simulink model "FOCwithLOAD"  (R2024b)
settings: Solver=FixedStepDiscrete  StartTime=0.0  StopTime=inf  RelTol=1e-3
PreLoadFcn:
  | % 自动加载同目录下的 linear_data.m，确保换机/首次打开可直接更新与编译
  | if ~evalin('base', 'exist(''Ts'',''var'') && exist(''pmsm'',''var'') && exist(''SMRC_I_Vsat_thresh'',''var'')')
  |     mdlDir_ = '';
  |     if bdIsLoaded('FOCwithLOAD'), mdlDir_ = fileparts(get_param('FOCwithLOAD', 'FileName')); end
  |     if isempty(mdlDir_), mdlDir_ = fileparts(which('FOCwithLOAD')); end
  |     if isempty(mdlDir_), mdlDir_ = pwd; end
  |     dataFile_ = fullfile(mdlDir_, 'linear_data.m');
  |     if isfile(dataFile_)
  |         assignin('base', 'linearDataFileTmp_', dataFile_);
  |         evalin('base', 'run(linearDataFileTmp_); clear linearDataFileTmp_');
  |     end
  |     clear mdlDir_ dataFile_
  | end
InitFcn:
  | % 自动加载同目录下的 linear_data.m，确保换机/首次打开可直接更新与编译
  | if ~evalin('base', 'exist(''Ts'',''var'') && exist(''pmsm'',''var'') && exist(''SMRC_I_Vsat_thresh'',''var'')')
  |     mdlDir_ = '';
  |     if bdIsLoaded('FOCwithLOAD'), mdlDir_ = fileparts(get_param('FOCwithLOAD', 'FileName')); end
  |     if isempty(mdlDir_), mdlDir_ = fileparts(which('FOCwithLOAD')); end
  |     if isempty(mdlDir_), mdlDir_ = pwd; end
  |     dataFile_ = fullfile(mdlDir_, 'linear_data.m');
  |     if isfile(dataFile_)
  |         assignin('base', 'linearDataFileTmp_', dataFile_);
  |         evalin('base', 'run(linearDataFileTmp_); clear linearDataFileTmp_');
  |     end
  |     clear mdlDir_ dataFile_
  | end
values from neighbouring files (symbols this model uses):
  a_hat = Kt_eff / (pmsm.J * omega_pu_base)    [linear_data.m]
  ADRC_B0 = 6055    [linear_data.m]
  ADRC_Wc = 3.2e-3    (= 0.0032)    [linear_data.m]
  ADRC_Wo = 30    [linear_data.m]
  alpha_ppc = exp(-lambda_ppc*Ts_speed)    [linear_data.m]
  b_hat = pmsm.B/pmsm.J    [linear_data.m]
  beta1 = single(2.0 * w_o)    [linear_data.m]
  beta2_sat_scale = 0.2    [linear_data.m]
  dataType = 'single'    [linear_data.m]
  gamma_reset = 0.9    [linear_data.m]
  inv_a_hat = 1/double(a_hat)    [linear_data.m]
  k_xi = 55    [linear_data.m]
  Kff = 0.98931745    [linear_data.m]
  lambda_ppc = 45    [linear_data.m]
  P_inf_const = 0.004    [linear_data.m]
  PI_params = mcb_SetControllerParameters(pmsm,inverter,PU_System,T_pwm,Ts,Ts_speed)    [linear_data.m]
  pmsm2 = pmsm    [linear_data.m]
  s_limit_sat = 0.9    [linear_data.m]
  speedRPM2mmps = pmlsm.mmps_per_rpm    [linear_data.m]
  target = mcb_SetProcessorDetails('F28379D',PWM_frequency)    [linear_data.m]
  Ts = T_pwm    (= 5e-05)    [linear_data.m]
  Ts_motor = T_pwm/2    (= 2.5e-05)    [linear_data.m]
  Ts_speed = 1*Ts    (= 5e-05)    [linear_data.m]
  w_o = single(200.0)    [linear_data.m]
  z2_limit = single(100.0)    [linear_data.m]
undefined symbols (not defined in the file or in its folder): DiscIntNeverNeededParam, Down, GPTRIP1SEL, GPTRIP2SEL, innerPI, inverter, inverter2, outerPI, pmlsm, pmsm, Tctr, TZ1, TZ2, Up
libraries: c2802xlib x13, simulink x10, c2837xDlib x6, c280xlib x6, slpidlib x5, svdschedulerlib x4, mcbcontrolslib x4, mcbpositiondecoderlib x2, mcbpmsmnonlinearlib x2, autolibpmsmexterior x2, mcbplantlib x2, svdutilitieslib x1
(part 4 of 5)

== system FOCwithLOAD/Motor1 Speed control/Control_System/Closed Loop Control1/Controller ==
  iD_fdbk : Inport
  iQ_fdbk : Inport  Port=2
  IdqRef : Inport  Port=3
  dx_mm : Inport  Port=4
  EnSMRC_I : Inport  Port=5
  AlignModeReadQ : DataStoreRead  DataStoreName=AlignMode  IndexOptions=Index vector (dialog)  Indices=1  OutputSizes=1
  Demux : Demux  Outputs=2
  Inner D axis Controller : Subsystem
  Inner Q axis Controller : Subsystem
  IqFdbkAlignSw : Switch  Criteria=u2 > Threshold  Threshold=0.5  SaturateOnIntegerOverflow=off  InputSameDT=off
  VqAlignSw : Switch  Criteria=u2 > Threshold  Threshold=0.5  SaturateOnIntegerOverflow=off  InputSameDT=off
  ZeroSingleQ : Constant  Value=0  OutDataTypeStr=single
  uD_req : Outport
  uQ_req : Outport  Port=2
  wires:
  iD_fdbk/1 -> Inner D axis Controller/2(iD_fdbk)
  IdqRef/1 -> Demux/1
  Demux/1 -> Inner D axis Controller/1(iD_req)
  Demux/2 -> Inner Q axis Controller/1(iQ_req)
  Inner D axis Controller/1(uD_req) -> uD_req/1  "uD_req"
  VqAlignSw/1 -> uQ_req/1
  Inner Q axis Controller/1(uQ_req) -> VqAlignSw/3  "uQ_req"
  IqFdbkAlignSw/1 -> Inner Q axis Controller/2(iQ_fdbk)
  iQ_fdbk/1 -> IqFdbkAlignSw/3
  AlignModeReadQ/1 -> IqFdbkAlignSw/2, VqAlignSw/2
  ZeroSingleQ/1 -> IqFdbkAlignSw/1, VqAlignSw/1

== system FOCwithLOAD/Motor1 Speed control/Control_System/Closed Loop Control1/SVPWM ==
  note: 零序分量注入
  u_alpha : Inport
  u_beta : Inport  Port=2
  VBus : Inport  Port=3
  Constant : Constant
  Constant3 : Constant  Commented=on  Value=0.5  OutDataTypeStr=single
  Divide1 : Product  Commented=on  Inputs=*/
  Gain : Gain  Gain=2/Ts
  InvClark : Subsystem  Commented=on
  Scope : Scope
  Scope1 : Scope
  Sector Caculate : Subsystem
  Subtract : Sum  Inputs=+-  OutDataTypeStr=single
  Sum : Sum  Commented=on  Inputs=++|
  Sum2 : Sum  Commented=on  Inputs=|++
  T1T1 Caculate : Subsystem
  Tcm Caculate : Subsystem
  Tpwm : Constant  Value=Ts  OutDataTypeStr=double
  XYZ Caculate : Subsystem
  ei_t : Subsystem  Commented=on
  DutyABC : Outport
  wires:
  Constant3/1 -> Sum2/2
  Divide1/1 -> Sum2/1
  InvClark/1(u_abc_spwm) -> ei_t/1(u_abc_spwm), Sum/2  "spwm"
  ei_t/1(sit) -> Sum/1  "eit"
  Sum/1 -> Divide1/1
  u_beta/1 -> InvClark/2(u_beta), XYZ Caculate/2(Ubeta), Sector Caculate/2(Ubeta)
  u_alpha/1 -> InvClark/1(u_alpha), Sector Caculate/1(Ualpha), XYZ Caculate/1(Ualpha)
  VBus/1 -> XYZ Caculate/4(Udc), Divide1/2
  Constant/1 -> Subtract/1
  Tcm Caculate/1(Tcm1 Tcm2 Tcm3) -> Scope1/1, Gain/1
  T1T1 Caculate/2(T2) -> Tcm Caculate/3(T2)
  XYZ Caculate/1(XYZ) -> T1T1 Caculate/2(XYZ)
  Gain/1 -> Subtract/2
  Sector Caculate/1("N ") -> Tcm Caculate/1(N), T1T1 Caculate/1(N)
  Tpwm/1 -> XYZ Caculate/3(Ts), Tcm Caculate/4(Tpwm), T1T1 Caculate/3(Tpwm)
  T1T1 Caculate/1(T1) -> Tcm Caculate/2(T1)
  Subtract/1 -> DutyABC/1, Scope/1

== system FOCwithLOAD/Motor1 Speed control/Control_System/Closed Loop Control1/Sample Choice ==
  note: 在电流采样中，ADC在mosfet导通时，进行电压测算，反推出电流，
      | 当上桥臂极高占空比时，导致下桥臂占空比极低，测量时间极短。
      | 开关噪声等会影响测量。
      |
      | 判断占空比大小，选用合适的下桥臂电流进行计算。Ia+Ib+Ic=0
  Duty : Inport
  Iabc : Inport  Port=2
  AB 采样计算2 : Subsystem  TreatAsAtomicUnit=on
  AC 采样计算1 : Subsystem  TreatAsAtomicUnit=on
  BC 采样计算 : Subsystem  TreatAsAtomicUnit=on
  Demux1 : Demux  Outputs=3
  If : If  NumInputs=3  IfExpression=u1 >= u2 & u1 >= u3  ElseIfExpressions=u2 >= u1 & u2 >= u3
  Merge : Merge  Inputs=3
  IABC : Outport
  wires:
  If/1 -> BC 采样计算/Action  "BC采样"
  Iabc/1 -> BC 采样计算/1(Iabc), AB 采样计算2/1(Iabc), AC 采样计算1/1(Iabc)
  If/2 -> AC 采样计算1/Action  "AC采样"
  Duty/1 -> Demux1/1
  Demux1/1 -> If/1
  If/3 -> AB 采样计算2/Action  "AB采样"
  Merge/1 -> IABC/1
  BC 采样计算/1(IABC) -> Merge/1
  Demux1/3 -> If/3
  Demux1/2 -> If/2
  AC 采样计算1/1(IABC) -> Merge/2
  AB 采样计算2/1(IABC) -> Merge/3

== system FOCwithLOAD/Motor1 Speed control/Control_System/Closed Loop Control1/clark ==
  note: $i_\alpha=\frac{2}{3}i_a-\frac{1}{3}(i_b+i_c) \\ i_\beta=\frac{\sqrt{3}}{3}(i_b-i_c)$
  i_a : Inport
  i_b : Inport  Port=2
  i_c : Inport  Port=3
  Gain : Gain  Gain=2/3
  Gain1 : Gain  Gain=1/3
  Gain2 : Gain  Gain=sqrt(3)/3
  Sum : Sum  Inputs=|++
  Sum1 : Sum  Inputs=|+-
  Sum2 : Sum  Inputs=+-|
  i_alpha : Outport
  i_beta : Outport  Port=2
  wires:
  Gain2/1 -> i_beta/1
  Sum2/1 -> Gain2/1
  Sum1/1 -> i_alpha/1
  Gain1/1 -> Sum1/2
  Gain/1 -> Sum1/1
  i_a/1 -> Gain/1
  i_c/1 -> Sum/2, Sum2/2
  Sum/1 -> Gain1/1
  i_b/1 -> Sum/1, Sum2/1

== system FOCwithLOAD/Motor1 Speed control/Control_System/Closed Loop Control1/inv_park ==
  note: $i_{\alpha} = i_d cos(\theta_e )- i_q sin(\theta_e )\\ i_{\beta} = i_d sin(\theta_e )+ i_q cos(\theta_e )$
  u_d : Inport
  u_q : Inport  Port=2
  sincos : Inport  Port=3
  Add : Sum  Inputs=+-
  Add1 : Sum
  Demux : Demux  Outputs=2
  Product{,1..3} (4 alike) : Product
  u_alpha : Outport
  u_beta : Outport  Port=2
  wires:
  sincos/1 -> Demux/1
  Demux/2 -> Product3/2, Product/2
  Demux/1 -> Product2/2, Product1/2
  Add1/1 -> u_beta/1
  Product3/1 -> Add1/2
  Product2/1 -> Add1/1
  Add/1 -> u_alpha/1
  Product1/1 -> Add/2
  u_q/1 -> Product1/1, Product3/1
  Product/1 -> Add/1
  u_d/1 -> Product/1, Product2/1  "i_d"

== system FOCwithLOAD/Motor1 Speed control/Control_System/Closed Loop Control1/park ==
  note: $i_{d} = i_{\alpha} cos(\theta_e )+ i_{\beta} sin(\theta_e ) \\ i_{q} = -i_{\alpha} sin(\theta_e )+ i_{\beta} cos(\theta_e )$
  i_alpha : Inport
  i_beta : Inport  Port=2
  sincos : Inport  Port=3
  Demux : Demux  Outputs=2
  Product{,1..3} (4 alike) : Product
  Sum : Sum  Inputs=|++
  Sum1 : Sum  Inputs=|-+
  i_d : Outport
  i_q : Outport  Port=2
  wires:
  sincos/1 -> Demux/1
  Sum1/1 -> i_q/1
  Product3/1 -> Sum1/2
  Product2/1 -> Sum1/1
  i_beta/1 -> Product1/1, Product3/1
  Sum/1 -> i_d/1
  Product1/1 -> Sum/2
  Product/1 -> Sum/1
  Demux/1 -> Product2/2, Product1/2  "sin"
  Demux/2 -> Product/2, Product3/2  "cos"
  i_alpha/1 -> Product/1, Product2/1

== system FOCwithLOAD/Motor1 Speed control/Input Scaling/ Calculate Position and Speed/PosDelta ==
  theta_pu : Inport
  C_Half : Constant  Value=single(0.5)
  C_InitOne : Constant  Value=single(1.0)
  C_One : Constant  Value=single(1.0)
  C_Zero : Constant  Value=single(0.0)
  Gain_mm : Gain  Gain=single(20.0)
  Mod_Wrap : Math  Operator=mod
  Sum_AddHalf : Sum
  Sum_Diff : Sum  Inputs=+-
  Sum_SubHalf : Sum  Inputs=+-
  Sw_Init : Switch  Criteria=u2 > Threshold  Threshold=0.5  SaturateOnIntegerOverflow=off  InputSameDT=off
  ToSingle : DataTypeConversion  OutDataTypeStr=single  SaturateOnIntegerOverflow=off  RndMeth=Floor
  UD_Init : UnitDelay  InitialCondition=single(0.0)  SampleTime=-1  HasFrameUpgradeWarning=on
  UD_Theta : UnitDelay  InitialCondition=single(0)  SampleTime=-1  HasFrameUpgradeWarning=on
  dx_mm : Outport
  wires:
  Sw_Init/1 -> dx_mm/1
  C_Zero/1 -> Sw_Init/3
  UD_Init/1 -> Sw_Init/2
  Gain_mm/1 -> Sw_Init/1
  C_InitOne/1 -> UD_Init/1
  Sum_SubHalf/1 -> Gain_mm/1
  Mod_Wrap/1 -> Sum_SubHalf/1
  C_One/1 -> Mod_Wrap/2
  Sum_AddHalf/1 -> Mod_Wrap/1
  C_Half/1 -> Sum_AddHalf/2, Sum_SubHalf/2
  Sum_Diff/1 -> Sum_AddHalf/1
  UD_Theta/1 -> Sum_Diff/2
  ToSingle/1 -> UD_Theta/1, Sum_Diff/1
  theta_pu/1 -> ToSingle/1

== system FOCwithLOAD/Motor1 Speed control/Input Scaling/Calculate Phase Currents/Data_Type ==
  In1 : Inport
  Data_Type_Fixed_Point : Subsystem  VariantControl=~isequal(dataType,'single')
  Data_Type_Float : Subsystem  VariantControl=isequal(dataType,'single')
  Iabc_meas_Real : Outport

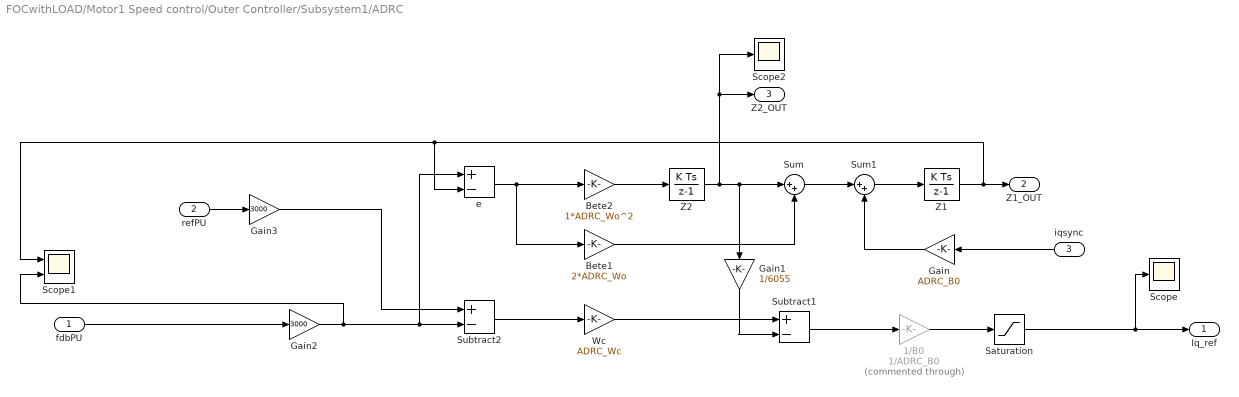
== system FOCwithLOAD/Motor1 Speed control/Outer Controller/Subsystem1/ADRC ==
  fdbPU : Inport
  refPU : Inport  Port=2
  iqsync : Inport  Port=3
  1/B0 : Gain  Commented=through  Gain=1/ADRC_B0
  Bete1 : Gain  Gain=2*ADRC_Wo
  Bete2 : Gain  Gain=1*ADRC_Wo^2
  Gain : Gain  Gain=ADRC_B0
  Gain1 : Gain  Gain=1/6055
  Gain2 : Gain  Gain=3000
  Gain3 : Gain  Gain=3000
  Saturation : Saturate  UpperLimit=8  LowerLimit=-8
  Scope : Scope
  Scope1 : Scope  NumInputPorts=2
  Scope2 : Scope
  Subtract1 : Sum  Inputs=+-
  Subtract2 : Sum  Inputs=+-
  Sum : Sum  Inputs=|++
  Sum1 : Sum  Inputs=|++
  Wc : Gain  Gain=ADRC_Wc
  Z1 : DiscreteIntegrator  SampleTime=-1  ICPrevOutput=DiscIntNeverNeededParam  ICPrevScaledInput=DiscIntNeverNeededParam
  Z2 : DiscreteIntegrator  SampleTime=-1  ICPrevOutput=DiscIntNeverNeededParam  ICPrevScaledInput=DiscIntNeverNeededParam
  e : Sum  Inputs=+-
  Iq_ref : Outport
  Z1_OUT : Outport  Port=2
  Z2_OUT : Outport  Port=3
  wires:
  e/1 -> Bete1/1, Bete2/1
  Bete2/1 -> Z2/1
  Bete1/1 -> Sum/2
  Sum/1 -> Sum1/1
  Wc/1 -> Subtract1/1
  Subtract2/1 -> Wc/1
  Subtract1/1 -> 1/B0/1
  1/B0/1 -> Saturation/1
  Z2/1 -> Scope2/1, Z2_OUT/1, Sum/1, Gain1/1
  Sum1/1 -> Z1/1
  Z1/1 -> Z1_OUT/1, e/2, Scope1/1
  Saturation/1 -> Scope/1, Iq_ref/1
  iqsync/1 -> Gain/1
  refPU/1 -> Gain3/1
  Gain/1 -> Sum1/2
  Gain1/1 -> Subtract1/2
  Gain2/1 -> Scope1/2, e/1, Subtract2/2
  Gain3/1 -> Subtract2/1
  fdbPU/1 -> Gain2/1

== system FOCwithLOAD/Motor1 Speed control/Outer Controller/ppc/P_decay ==
  P_inf_const : Inport
  P_select : Inport  Port=2
  1 : Sum  Inputs=|++
  P_z1 : UnitDelay  SampleTime=-1  HasFrameUpgradeWarning=on
  PminusPinf : Sum  Inputs=|+-
  alpha_gain : Gain  Gain=alpha_ppc
  P_decay_sum : Outport
  wires:
  P_inf_const/1 -> PminusPinf/2, 1/2
  P_select/1 -> P_z1/1
  alpha_gain/1 -> 1/1
  1/1 -> P_decay_sum/1
  P_z1/1 -> PminusPinf/1
  PminusPinf/1 -> alpha_gain/1

== system FOCwithLOAD/Motor1 Speed control/Outer Controller/ppc/P_reset ==
  e_calc : Inport
  P_inf_const : Inport  Port=2
  Gain : Gain  Gain=1.25
  P_floor_sum : Sum  Inputs=|++
  P_reset_max : MinMax  Function=max  Inputs=2
  abs_e : Abs  SaturateOnIntegerOverflow=off
  eps_p_const : Constant  Value=0.001
  P_reset : Outport
  wires:
  P_floor_sum/1 -> P_reset_max/2
  abs_e/1 -> Gain/1
  eps_p_const/1 -> P_floor_sum/2
  Gain/1 -> P_reset_max/1
  P_reset_max/1 -> P_reset/1
  e_calc/1 -> abs_e/1
  P_inf_const/1 -> P_floor_sum/1

== system FOCwithLOAD/Motor1 Speed control/Outer Controller/ppc/eso ==
  Iq_ref_prev : Inport
  speed_fdbk : Inport  Port=2
  Abs : Abs  SaturateOnIntegerOverflow=off
  Compare To Constant : simulink/Logic and Bit Operations/Compare To Constant  relop=>  const=7.95  OutDataTypeStr=boolean
  Constant : Constant  Value=w_o * w_o
  Constant1 : Constant  Value=beta2_sat_scale * w_o * w_o
  Discrete-Time Integrator1 : DiscreteIntegrator  SampleTime=-1  ICPrevOutput=DiscIntNeverNeededParam  ICPrevScaledInput=DiscIntNeverNeededParam
  Gain1 : Gain  Gain=a_hat
  Gain2 : Gain  Gain=-beta1
  Gain3 : Gain  Gain=-b_hat
  Gain4 : Gain  Gain=-1
  Gain5 : Gain  Gain=Ts_speed
  Product : Product
  Saturation : Saturate  UpperLimit=z2_limit  LowerLimit=-z2_limit
  Sum : Sum  Inputs=++++
  Switch : Switch  Criteria=u2 ~= 0  SaturateOnIntegerOverflow=off  InputSameDT=off
  Unit Delay : UnitDelay  SampleTime=-1  HasFrameUpgradeWarning=on
  e : Sum  Inputs=|++
  e_obs : Sum  Inputs=|+-
  Z1 : Outport
  Z2 : Outport  Port=2
  wires:
  speed_fdbk/1 -> e_obs/2
  e_obs/1 -> Product/2, Gain2/1  "e_obs"
  Saturation/1 -> Sum/1, Z2/1, Unit Delay/1  "z2_next"
  Iq_ref_prev/1 -> Abs/1, Gain1/1
  Gain1/1 -> Sum/2
  Gain2/1 -> Sum/3
  Sum/1 -> Discrete-Time Integrator1/1
  Discrete-Time Integrator1/1 -> Gain3/1, Z1/1, e_obs/1
  Gain3/1 -> Sum/4
  Abs/1 -> Compare To Constant/1
  Compare To Constant/1 -> Switch/2
  Constant1/1 -> Switch/1
  Constant/1 -> Switch/3
  Product/1 -> Gain4/1
  Switch/1 -> Product/1
  Gain4/1 -> Gain5/1
  Gain5/1 -> e/1
  e/1 -> Saturation/1
  Unit Delay/1 -> e/2

== system FOCwithLOAD/Motor1 Speed control/Outer Controller/ppc/ref_jump_detect ==
  SpeedPU_req : Inport
  e__calc : Inport  Port=2
  p_select : Inport  Port=3
  Abs : Abs  SaturateOnIntegerOverflow=off
  Delay : Delay  DelayLength=1  InitialCondition=0
  Gain1 : Gain  Gain=gamma_reset
  GreaterThan : RelationalOperator  Operator=>  OutDataTypeStr=boolean  RndMeth=Simplest  InputSameDT=off
  Logical Operator : Logic  Operator=OR  AllPortsSameDT=off  OutDataTypeStr=boolean
  abs_dwref : Abs  SaturateOnIntegerOverflow=off
  delta_ref_const : Constant  Value=P_inf_const
  dwref_calc : Sum  Inputs=|+-
  ref_jump_detect : RelationalOperator  Operator=>  OutDataTypeStr=boolean  RndMeth=Simplest  InputSameDT=off
  wref_z1 : UnitDelay  SampleTime=-1  HasFrameUpgradeWarning=on
  output : Outport
  wires:
  dwref_calc/1 -> abs_dwref/1
  SpeedPU_req/1 -> dwref_calc/1, wref_z1/1
  abs_dwref/1 -> ref_jump_detect/1
  wref_z1/1 -> dwref_calc/2
  delta_ref_const/1 -> ref_jump_detect/2
  e__calc/1 -> Abs/1
  Gain1/1 -> GreaterThan/2
  Delay/1 -> Gain1/1
  p_select/1 -> Delay/1
  Abs/1 -> GreaterThan/1
  ref_jump_detect/1 -> Logical Operator/1
  GreaterThan/1 -> Logical Operator/2
  Logical Operator/1 -> output/1

== system FOCwithLOAD/Motor1 Speed control/Outer Controller/ppc/term1 ==
  e_calc : Inport
  P_select : Inport  Port=2
  P_inf_const : Inport  Port=3
  Pdot_over_P : Product  Inputs=*/
  PminusPinf_forPdot : Sum  Inputs=|+-
  neg_lambda_gain : Gain  Gain=-lambda_ppc
  term1_product : Product
  term1 : Outport
  wires:
  neg_lambda_gain/1 -> Pdot_over_P/1
  P_inf_const/1 -> PminusPinf_forPdot/2
  P_select/1 -> PminusPinf_forPdot/1, Pdot_over_P/2
  Pdot_over_P/1 -> term1_product/1
  PminusPinf_forPdot/1 -> neg_lambda_gain/1
  term1_product/1 -> term1/1
  e_calc/1 -> term1_product/2

== system FOCwithLOAD/Motor1 Speed control/Outer Controller/ppc/term2 ==
  P_select : Inport
  xi : Inport  Port=2
  s_limit_sat_1 : Inport  Port=3
  Constant : Constant
  Math Function : Math  Operator=square
  P_times_ones2 : Product
  Sum1 : Sum  Inputs=|+-
  kxi_gain : Gain  Gain=k_xi
  term2_product : Product
  Out1 : Outport
  wires:
  kxi_gain/1 -> term2_product/1
  P_select/1 -> P_times_ones2/1
  P_times_ones2/1 -> kxi_gain/1
  Sum1/1 -> P_times_ones2/2
  xi/1 -> term2_product/2
  term2_product/1 -> Out1/1
  s_limit_sat_1/1 -> Math Function/1
  Math Function/1 -> Sum1/2
  Constant/1 -> Sum1/1

== system FOCwithLOAD/Motor1 Speed control/Outer Controller/ppc/xi ==
  In1 : Inport
  Gain : Gain  Gain=0.5
  ln_ratio : Math  Operator=log
  one_const_blk : Constant
  one_minus_s : Sum  Inputs=|+-
  one_plus_s : Sum  Inputs=|++
  ratio_divide : Product  Inputs=*/
  s_limit_sat : Saturate  UpperLimit=s_limit_sat  LowerLimit=-s_limit_sat
  xi : Outport
  s_limit_sat_1 : Outport  Port=2
  wires:
  In1/1 -> s_limit_sat/1
  one_const_blk/1 -> one_minus_s/1, one_plus_s/1
  one_minus_s/1 -> ratio_divide/2
  ratio_divide/1 -> ln_ratio/1
  Gain/1 -> xi/1
  ln_ratio/1 -> Gain/1
  one_plus_s/1 -> ratio_divide/1
  s_limit_sat/1 -> s_limit_sat_1/1, one_minus_s/2, one_plus_s/2

== system FOCwithLOAD/Motor1 Speed control/SCI (Code Generation)/Data_Conditioning_Tx/Data_Type_Fixed_Point ==
  In1 : Inport
  Data Type Conversion : DataTypeConversion  OutDataTypeStr=fixdt(1,32,28)  RndMeth=Simplest  SaturateOnIntegerOverflow=off
  Data Type Conversion3 : DataTypeConversion  OutDataTypeStr=uint32  ConvertRealWorld=Stored Integer (SI)  RndMeth=Simplest  SaturateOnIntegerOverflow=off
  Data_Log : Outport
  wires:
  In1/1 -> Data Type Conversion/1
  Data Type Conversion3/1 -> Data_Log/1
  Data Type Conversion/1 -> Data Type Conversion3/1

== system FOCwithLOAD/Motor1 Speed control/SCI (Code Generation)/Data_Conditioning_Tx/Data_Type_Float ==
  In1 : Inport
  Byte Pack : svdutilitieslib/Byte Pack  maskPackedDataType=uint32  datatypes={'single'}  byteAlign=4  blockPlatform=tic2000
  Data_Log : Outport
  wires:
  Byte Pack/1 -> Data_Log/1
  In1/1 -> Byte Pack/1

== system FOCwithLOAD/Motor1 Speed control/SCI (Code Generation)/Data_Logging/Data ==
  Data : Inport
  Data_width : Inport  Port=2
  Action Port : ActionPort  ActionPortLabel=else
  Dummy : Constant  Value=hex2dec('0000')  OutDataTypeStr=uint32
  Mux : Mux  Inputs=2
  Data_out : Outport  VectorParamsAs1DForOutWhenUnconnected=off
  Iteration : Outport  Port=2  VectorParamsAs1DForOutWhenUnconnected=off
  wires:
  Data_width/1 -> Iteration/1
  Data/1 -> Mux/1
  Dummy/1 -> Mux/2
  Mux/1 -> Data_out/1

== system FOCwithLOAD/Motor1 Speed control/SCI (Code Generation)/Data_Logging/End ==
  Data : Inport
  Data_width : Inport  Port=2
  Action Port : ActionPort  ActionPortLabel=elseif(u1 == 599)
  Bias : Bias  Bias=1  SaturateOnIntegerOverflow=off
  End : Constant  Value=hex2dec('45454545')  OutDataTypeStr=uint32
  Mux : Mux  Inputs=2
  Data_out : Outport  VectorParamsAs1DForOutWhenUnconnected=off
  Iteration : Outport  Port=2  VectorParamsAs1DForOutWhenUnconnected=off
  wires:
  Data/1 -> Mux/1
  Data_width/1 -> Bias/1
  Bias/1 -> Iteration/1
  End/1 -> Mux/2
  Mux/1 -> Data_out/1

== system FOCwithLOAD/Motor1 Speed control/SCI (Code Generation)/Data_Logging/Start ==
  Data : Inport
  Data_width : Inport  Port=2
  Action Port : ActionPort  ActionPortLabel=if(u1 == 0)
  Bias : Bias  Bias=1  SaturateOnIntegerOverflow=off
  Mux : Mux  Inputs=2
  Start : Constant  Value=hex2dec('53535353')  OutDataTypeStr=uint32
  Data_out : Outport  VectorParamsAs1DForOutWhenUnconnected=off
  Iteration : Outport  Port=2  VectorParamsAs1DForOutWhenUnconnected=off
  wires:
  Data/1 -> Mux/2
  Data_width/1 -> Bias/1
  Bias/1 -> Iteration/1
  Start/1 -> Mux/1
  Mux/1 -> Data_out/1

== system FOCwithLOAD/Motor1 and Motor2 coupled/Simulation/Motor1_Measurements/Get_PU  ==
  rad : Inport
  Constant2 : Constant  Value=2*pi  OutDataTypeStr=single  SampleTime=-1
  Get_PU : Gain  Gain=1/(2*pi)  RndMeth=Simplest  OutDataTypeStr=Inherit: Same as input
  Mod : Math  Operator=mod
  PU : Outport  VectorParamsAs1DForOutWhenUnconnected=off
  wires:
  Get_PU/1 -> PU/1
  Mod/1 -> Get_PU/1
  Constant2/1 -> Mod/2
  rad/1 -> Mod/1

== system FOCwithLOAD/Motor1 and Motor2 coupled/Simulation/Motor1_Measurements/Wrap ==
  in : Inport
  Constant2 : Constant  OutDataTypeStr=single  SampleTime=-1
  Mod : Math  Operator=mod
  out : Outport  VectorParamsAs1DForOutWhenUnconnected=off
  wires:
  Mod/1 -> out/1
  Constant2/1 -> Mod/2
  in/1 -> Mod/1

== system FOCwithLOAD/Motor1 and Motor2 coupled/Simulation/Motor2_Measurements/Get_PU  ==
  rad : Inport
  Constant2 : Constant  Value=2*pi  OutDataTypeStr=single  SampleTime=-1
  Get_PU : Gain  Gain=1/(2*pi)  RndMeth=Simplest  OutDataTypeStr=Inherit: Same as input
  Mod : Math  Operator=mod
  PU : Outport  VectorParamsAs1DForOutWhenUnconnected=off
  wires:
  rad/1 -> Mod/1
  Constant2/1 -> Mod/2
  Mod/1 -> Get_PU/1
  Get_PU/1 -> PU/1

== system FOCwithLOAD/Motor1 and Motor2 coupled/Simulation/Motor2_Measurements/Wrap ==
  in : Inport
  Constant2 : Constant  OutDataTypeStr=single  SampleTime=-1
  Mod : Math  Operator=mod
  out : Outport  VectorParamsAs1DForOutWhenUnconnected=off
  wires:
  in/1 -> Mod/1
  Constant2/1 -> Mod/2
  Mod/1 -> out/1

== system FOCwithLOAD/Motor2 Torque control/Control_System/Closed Loop Control1/Angle Compensate ==
  ThetaeSample : Inport
  SpeedSample : Inport  Port=2
  Add : Sum
  Gain : Gain  Gain=pmsm2.p/(60*speedRPM2mmps)*Ts
  Thetae : Outport
  wires:
  Gain/1 -> Add/2
  Add/1 -> Thetae/1
  SpeedSample/1 -> Gain/1
  ThetaeSample/1 -> Add/1

== system FOCwithLOAD/Motor2 Torque control/Control_System/Closed Loop Control1/Controller ==
  iD_fdbk : Inport
  iQ_fdbk : Inport  Port=2
  IdqRef : Inport  Port=3
  AlignMode2ReadQ : DataStoreRead  DataStoreName=AlignMode2  IndexOptions=Index vector (dialog)  Indices=1  OutputSizes=1
  Demux : Demux  Outputs=2
  Filter : Subsystem  Commented=on
  Filter1 : Subsystem  Commented=on
  Inner D axis Controller : Subsystem
  Inner Q axis Controller : Subsystem
  IqFdbkAlignSw2 : Switch  Criteria=u2 > Threshold  Threshold=0.5  SaturateOnIntegerOverflow=off  InputSameDT=off
  VqAlignSw2 : Switch  Criteria=u2 > Threshold  Threshold=0.5  SaturateOnIntegerOverflow=off  InputSameDT=off
  ZeroSingleQ2 : Constant  Value=0  OutDataTypeStr=single
  uD_req : Outport
  uQ_req : Outport  Port=2
  wires:
  IdqRef/1 -> Demux/1
  Demux/1 -> Inner D axis Controller/1(iD_req)
  Demux/2 -> Inner Q axis Controller/1(iQ_req)
  Inner D axis Controller/1(uD_req) -> uD_req/1  "uD_req"
  iD_fdbk/1 -> Inner D axis Controller/2(iD_fdbk)
  ? -> Filter1/1(R(n))
  ? -> Filter/1(R(n))
  VqAlignSw2/1 -> uQ_req/1
  Inner Q axis Controller/1(uQ_req) -> VqAlignSw2/3  "uQ_req"
  IqFdbkAlignSw2/1 -> Inner Q axis Controller/2(iQ_fdbk)
  iQ_fdbk/1 -> IqFdbkAlignSw2/3
  AlignMode2ReadQ/1 -> VqAlignSw2/2, IqFdbkAlignSw2/2
  ZeroSingleQ2/1 -> IqFdbkAlignSw2/1, VqAlignSw2/1

== system FOCwithLOAD/Motor2 Torque control/Control_System/Closed Loop Control1/SVPWM ==
  note: 相电压+三次谐波补偿=Uabc-母线电压的一半
  u_alpha : Inport
  u_beta : Inport  Port=2
  VBus : Inport  Port=3
  Constant3 : Constant  Value=0.5  OutDataTypeStr=single
  Divide1 : Product  Inputs=*/
  InvClark : Subsystem
  Sum : Sum  Inputs=++|
  Sum2 : Sum  Inputs=|++
  ei_t : Subsystem
  DutyABC : Outport
  wires:
  Sum2/1 -> DutyABC/1  "占空比"
  Constant3/1 -> Sum2/2
  Divide1/1 -> Sum2/1
  VBus/1 -> Divide1/2
  InvClark/1(u_abc_spwm) -> ei_t/1(u_abc_spwm), Sum/2  "spwm"
  ei_t/1(sit) -> Sum/1  "eit"
  u_beta/1 -> InvClark/2(u_beta)
  u_alpha/1 -> InvClark/1(u_alpha)
  Sum/1 -> Divide1/1

== system FOCwithLOAD/Motor2 Torque control/Control_System/Closed Loop Control1/Sample Choice ==
  Duty : Inport
  Iabc : Inport  Port=2
  AB 采样计算2 : Subsystem  TreatAsAtomicUnit=on
  AC 采样计算1 : Subsystem  TreatAsAtomicUnit=on
  BC 采样计算 : Subsystem  TreatAsAtomicUnit=on
  Demux1 : Demux  Outputs=3
  If : If  NumInputs=3  IfExpression=u1 >= u2 & u1 >= u3  ElseIfExpressions=u2 >= u1 & u2 >= u3
  Merge : Merge  Inputs=3
  IABC : Outport
  wires:
  If/1 -> BC 采样计算/Action  "BC采样"
  Iabc/1 -> BC 采样计算/1(Iabc), AB 采样计算2/1(Iabc), AC 采样计算1/1(Iabc)
  If/2 -> AC 采样计算1/Action  "AC采样"
  Duty/1 -> Demux1/1
  Demux1/1 -> If/1
  If/3 -> AB 采样计算2/Action  "AB采样"
  Merge/1 -> IABC/1
  BC 采样计算/1(IABC) -> Merge/1
  Demux1/3 -> If/3
  Demux1/2 -> If/2
  AC 采样计算1/1(IABC) -> Merge/2
  AB 采样计算2/1(IABC) -> Merge/3

== system FOCwithLOAD/Motor2 Torque control/Control_System/Closed Loop Control1/clark ==
  note: $i_\alpha=\frac{2}{3}i_a-\frac{1}{3}(i_b+i_c) \\ i_\beta=\frac{\sqrt{3}}{3}(i_b-i_c)$
  i_a : Inport
  i_b : Inport  Port=2
  i_c : Inport  Port=3
  Gain : Gain  Gain=2/3
  Gain1 : Gain  Gain=1/3
  Gain2 : Gain  Gain=sqrt(3)/3
  Sum : Sum  Inputs=|++
  Sum1 : Sum  Inputs=|+-
  Sum2 : Sum  Inputs=+-|
  i_alpha : Outport
  i_beta : Outport  Port=2
  wires:
  Gain2/1 -> i_beta/1
  Sum2/1 -> Gain2/1
  Sum1/1 -> i_alpha/1
  Gain1/1 -> Sum1/2
  Gain/1 -> Sum1/1
  i_a/1 -> Gain/1
  i_c/1 -> Sum/2, Sum2/2
  Sum/1 -> Gain1/1
  i_b/1 -> Sum/1, Sum2/1

== system FOCwithLOAD/Motor2 Torque control/Control_System/Closed Loop Control1/inv_park ==
  note: $i_{\alpha} = i_d cos(\theta_e )- i_q sin(\theta_e )\\ i_{\beta} = i_d sin(\theta_e )+ i_q cos(\theta_e )$
  u_d : Inport
  u_q : Inport  Port=2
  sincos : Inport  Port=3
  Add : Sum  Inputs=+-
  Add1 : Sum
  Demux : Demux  Outputs=2
  Product{,1..3} (4 alike) : Product
  u_alpha : Outport
  u_beta : Outport  Port=2
  wires:
  sincos/1 -> Demux/1
  Demux/2 -> Product3/2, Product/2
  Demux/1 -> Product2/2, Product1/2
  Add1/1 -> u_beta/1
  Product3/1 -> Add1/2
  Product2/1 -> Add1/1
  Add/1 -> u_alpha/1
  Product1/1 -> Add/2
  u_q/1 -> Product1/1, Product3/1
  Product/1 -> Add/1
  u_d/1 -> Product/1, Product2/1  "i_d"

== system FOCwithLOAD/Motor2 Torque control/Control_System/Closed Loop Control1/park ==
  note: $i_{d} = i_{\alpha} cos(\theta_e )+ i_{\beta} sin(\theta_e ) \\ i_{q} = -i_{\alpha} sin(\theta_e )+ i_{\beta} cos(\theta_e )$
  i_alpha : Inport
  i_beta : Inport  Port=2
  sincos : Inport  Port=3
  Demux : Demux  Outputs=2
  Product{,1..3} (4 alike) : Product
  Sum : Sum  Inputs=|++
  Sum1 : Sum  Inputs=|-+
  i_d : Outport
  i_q : Outport  Port=2
  wires:
  sincos/1 -> Demux/1
  Sum1/1 -> i_q/1
  Product3/1 -> Sum1/2
  Product2/1 -> Sum1/1
  i_beta/1 -> Product1/1, Product3/1
  Sum/1 -> i_d/1
  Product1/1 -> Sum/2
  Product/1 -> Sum/1
  Demux/1 -> Product2/2, Product1/2  "sin"
  Demux/2 -> Product/2, Product3/2  "cos"
  i_alpha/1 -> Product/1, Product2/1

== system FOCwithLOAD/Motor2 Torque control/Input Scaling/Calculate Phase Currents/Data_Type ==
  In1 : Inport
  Data_Type_Fixed_Point : Subsystem  VariantControl=~isequal(dataType,'single')
  Data_Type_Float : Subsystem  VariantControl=isequal(dataType,'single')
  Iabc_meas_Real : Outport

== system FOCwithLOAD/Serial Receive/Parse SCI Rx/Data_Conditioning_Rx/Data_Type_Fixed_Point ==
  Rx : Inport
  Data Type Conversion1 : DataTypeConversion  OutDataTypeStr=dataType  RndMeth=Simplest  SaturateOnIntegerOverflow=off
  Data Type Conversion2 : DataTypeConversion  OutDataTypeStr=fixdt(1,32,28)  ConvertRealWorld=Stored Integer (SI)  RndMeth=Simplest  SaturateOnIntegerOverflow=off
  Data Type Conversion3 : DataTypeConversion  OutDataTypeStr=uint16  RndMeth=Simplest  SaturateOnIntegerOverflow=off
  Data Type Conversion4 : DataTypeConversion  OutDataTypeStr=dataType  RndMeth=Simplest  SaturateOnIntegerOverflow=off
  Data Type Conversion5 : DataTypeConversion  OutDataTypeStr=fixdt(1,32,28)  ConvertRealWorld=Stored Integer (SI)  RndMeth=Simplest  SaturateOnIntegerOverflow=off
  Demux : Demux  Outputs=3
  Desired Speed : Outport
  Out2 : Outport  Port=2
  Desired torque : Outport  Port=3
  wires:
  Rx/1 -> Demux/1
  Data Type Conversion1/1 -> Desired Speed/1
  Data Type Conversion2/1 -> Data Type Conversion1/1
  Demux/1 -> Data Type Conversion2/1
  Demux/2 -> Data Type Conversion3/1
  Data Type Conversion3/1 -> Out2/1
  Demux/3 -> Data Type Conversion5/1
  Data Type Conversion5/1 -> Data Type Conversion4/1
  Data Type Conversion4/1 -> Desired torque/1

== system FOCwithLOAD/Serial Receive/Parse SCI Rx/Data_Conditioning_Rx/Data_Type_Float ==
  Rx : Inport
  Data Type Conversion2 : DataTypeConversion  OutDataTypeStr=uint16  RndMeth=Simplest  SaturateOnIntegerOverflow=off
  Demux : Demux  Outputs=3
  Desired Speed : Outport
  Out2 : Outport  Port=2
  Desired torque : Outport  Port=3
  wires:
  Rx/1 -> Demux/1
  Demux/1 -> Desired Speed/1
  Data Type Conversion2/1 -> Out2/1
  Demux/2 -> Data Type Conversion2/1
  Demux/3 -> Desired torque/1

== system FOCwithLOAD/Serial Receive/Serial Receive/Serial Rx/Data_Type_Fixed_Point ==
  SCI Receive : c280xlib/SCI Receive  sciModule=A  dataHead=[170 85]  headerCheckMaxCount=32  dataTail=[85 170]  dataType=uint32  dataLenOptions=Length via dialog  dataDim=3  maxDataLength=1  initValue=0  errOption=Output the last received value  errValue=0  sampleTime=-1  blockingMode=on  timeOut=0.001  outputStatus=off
  Rx : Outport
  wires:
  SCI Receive/1 -> Rx/1

== system FOCwithLOAD/Serial Receive/Serial Receive/Serial Rx/Data_Type_Float ==
  SCI Receive : c280xlib/SCI Receive  sciModule=A  dataHead=[170 85]  headerCheckMaxCount=32  dataTail=[85 170]  dataType=single  dataLenOptions=Length via dialog  dataDim=3  maxDataLength=1  initValue=0  errOption=Output the last received value  errValue=0  sampleTime=-1  blockingMode=on  timeOut=0.001  outputStatus=off
  Rx : Outport
  wires:
  SCI Receive/1 -> Rx/1

== system FOCwithLOAD/Serial Receive/Signal Packing/Data_Conditioning_Tx/Data_Type_Fixed_Point ==
  Speedref : Inport
  In2 : Inport  Port=2
  IqRef : Inport  Port=3
  Data Type Conversion : DataTypeConversion  OutDataTypeStr=fixdt(1,32,28)  RndMeth=Simplest  SaturateOnIntegerOverflow=off
  Data Type Conversion1 : DataTypeConversion  OutDataTypeStr=uint32  RndMeth=Simplest  SaturateOnIntegerOverflow=off
  Data Type Conversion2 : DataTypeConversion  OutDataTypeStr=fixdt(1,32,28)  RndMeth=Simplest  SaturateOnIntegerOverflow=off
  Data Type Conversion3 : DataTypeConversion  OutDataTypeStr=uint32  ConvertRealWorld=Stored Integer (SI)  RndMeth=Simplest  SaturateOnIntegerOverflow=off
  Data Type Conversion4 : DataTypeConversion  OutDataTypeStr=uint32  ConvertRealWorld=Stored Integer (SI)  RndMeth=Simplest  SaturateOnIntegerOverflow=off
  Mux : Mux  Inputs=3
  Data : Outport
  wires:
  Speedref/1 -> Data Type Conversion/1
  Data Type Conversion3/1 -> Mux/1
  Data Type Conversion/1 -> Data Type Conversion3/1
  In2/1 -> Data Type Conversion1/1
  Data Type Conversion1/1 -> Mux/2
  Mux/1 -> Data/1
  Data Type Conversion2/1 -> Data Type Conversion4/1
  Data Type Conversion4/1 -> Mux/3
  IqRef/1 -> Data Type Conversion2/1

== system FOCwithLOAD/Serial Receive/Signal Packing/Data_Conditioning_Tx/Data_Type_Float ==
  Speedref : Inport
  In2 : Inport  Port=2
  IqRef : Inport  Port=3
  Data Type Conversion2 : DataTypeConversion  OutDataTypeStr=single  RndMeth=Simplest  SaturateOnIntegerOverflow=off
  Mux : Mux  Inputs=3
  Data : Outport
  wires:
  Speedref/1 -> Mux/1
  Mux/1 -> Data/1
  In2/1 -> Data Type Conversion2/1
  Data Type Conversion2/1 -> Mux/2
  IqRef/1 -> Mux/3

== system FOCwithLOAD/Motor1 Speed control/Control_System/Closed Loop Control1/Controller/Inner D axis Controller ==
  iD_req : Inport
  iD_fdbk : Inport  Port=2
  Constant1 : Constant  Value=innerPI.iD.Discrete.Kp  OutDataTypeStr=single
  Constant2 : Constant  Value=innerPI.iD.Discrete.KiTctr  OutDataTypeStr=single
  Constant6 : Constant  Value=0  OutDataTypeStr=single
  Discrete PI Controller with anti-windup & reset : slpidlib/PID Controller  Controller=PI  Form=Parallel  TimeDomain=Discrete-time  UseExternalTs=off  SampleTime=-1  IntegratorMethod=Forward Euler  FilterMethod=Forward Euler  ControllerParametersSource=external  P=1  I=1  UseKiTs=on  D=0  UseExternalDerivativeSource=off  N=100  UseFilter=on  TunerSelectOption=Transfer Function Based (PID Tuner App)  InitialConditionSource=external  InitialConditionForIntegrator=0  InitialConditionForFilter=0  DifferentiatorICPrevScaledInput=0  ExternalReset=none  TrackingMode=off  Kt=1  LimitOutput=on  SatLimitsSource=internal  UpperSaturationLimit=0.8*inverter.V_dc*sqrt(3)/3  LowerSaturationLimit=-0.8*inverter.V_dc*sqrt(3)/3  LinearizeAsGain=on  AntiWindupMode=clamping  Kb=1  LimitIntegrator=off  UpperIntegratorSaturationLimit=inf  LowerIntegratorSaturationLimit=-inf  RndMeth=Simplest  POutMin=[]  POutMax=[]  IOutMin=[]  IOutMax=[]  DOutMin=[]  DOutMax=[]  NOutMin=[]  NOutMax=[]  SumOutMin=[]  SumOutMax=[]  SaturationOutDataTypeStr=Inherit: Inherit via back propagation  SaturationOutMin=[]  SaturationOutMax=[]  PParamMin=[]  PParamMax=[]  IParamMin=[]  IParamMax=[]  DParamMin=[]  DParamMax=[]  NParamMin=[]  NParamMax=[]  KbParamMin=[]  KbParamMax=[]  KtParamMin=[]  KtParamMax=[]  KbOutMin=[]  KbOutMax=[]  KtOutMin=[]  KtOutMax=[]  IntegratorOutMin=[]  IntegratorOutMax=[]  FilterOutMin=[]  FilterOutMax=[]  SumI1OutMin=[]  SumI1OutMax=[]  SumI2OutMin=[]  SumI2OutMax=[]  SumI3OutMin=[]  SumI3OutMax=[]  SumI4OutMin=[]  SumI4OutMax=[]  SumDOutMin=[]  SumDOutMax=[]  DifferentiatorOutMin=[]  DifferentiatorOutMax=[]  FilterDiffOutCoefMin=[]  FilterDiffOutCoefMax=[]  ReciprocalOutMin=[]  ReciprocalOutMax=[]  SumDenOutMin=[]  SumDenOutMax=[]  SumNumOutMin=[]  SumNumOutMax=[]  DivideOutMin=[]  DivideOutMax=[]  UdiffTsProdOutMin=[]  UdiffTsProdOutMax=[]  NTsProdOutMin=[]  NTsProdOutMax=[]  UintegralTsProdOutMin=[]  UintegralTsProdOutMax=[]  UngainTsProdOutMin=[]  UngainTsProdOutMax=[]  ClampingZeroOutDataTypeStr=Inherit: Inherit via back propagation  ClampingZeroOutMin=[]  ClampingZeroOutMax=[]  FilterDenConstantOutDataTypeStr=Inherit: Inherit via back propagation  FilterDenConstantOutMin=[]  FilterDenConstantOutMax=[]  PCopyOutDataTypeStr=Inherit: Inherit via back propagation  PCopyOutMin=[]  PCopyOutMax=[]  NCopyOutDataTypeStr=Inherit: Inherit via back propagation  NCopyOutMin=[]  NCopyOutMax=[]  IntegratorContinuousStateAttributes=''  IntegratorStateMustResolveToSignalObject=off  IntegratorRTWStateStorageClass=Auto  FilterContinuousStateAttributes=''  FilterStateMustResolveToSignalObject=off  FilterRTWStateStorageClass=Auto  ParallelPVariant=ExternalParameters  IdealPVariant=Disabled  IVariant=ExternalParameters  DVariant=Disabled  IntegratorVariant=Discrete  SatVariant=Enabled  AWVariant=DiscClampingParallel  PCopyVariant=Disabled  TRVariant=Disabled  FdbkBlocksVariant=Forward  IdealPFdbkVariant=Disabled  SatFdbkVariant=Disabled  DerivativeFilterVariant=Disabled  NVariant=Disabled  NCopyVariant=Disabled_SignalSpec  FilterICVariant=Disabled  IntegratorICVariant=ExternalICs  ExternalResetVariant=Disabled  TRSumVariant=Passthrough  SumFdbkVariant=Disabled  SumVariant=Sum_PI  TsampFilterVariant=InternalTs  TsampNgainVariant=Passthrough  TsampIntegralVariant=Disabled_SignalSpec  ExternalSaturationOutDataTypeStr=Inherit: Same as second input  DerivativeSourceVariant=Disabled  PreIntVariant=InternalPreInt
      settings: LibrarySourceBlock=mcbcontrolslib/PI Controller
  Sum1 : Sum  Inputs=|+-
  uD_req : Outport
  wires:
  Constant6/1 -> Discrete PI Controller with anti-windup & reset/4
  Discrete PI Controller with anti-windup & reset/1 -> uD_req/1
  Constant2/1 -> Discrete PI Controller with anti-windup & reset/3
  Constant1/1 -> Discrete PI Controller with anti-windup & reset/2
  iD_fdbk/1 -> Sum1/2
  iD_req/1 -> Sum1/1
  Sum1/1 -> Discrete PI Controller with anti-windup & reset/1

== system FOCwithLOAD/Motor1 Speed control/Control_System/Closed Loop Control1/Controller/Inner Q axis Controller ==
  iQ_req : Inport
  iQ_fdbk : Inport  Port=2
  Constant1 : Constant  Value=innerPI.iQ.Discrete.KiTctr  OutDataTypeStr=single
  Constant2 : Constant  Value=innerPI.iQ.Discrete.Kp  OutDataTypeStr=single
  Constant6 : Constant  Value=0  OutDataTypeStr=single
  Discrete PI Controller with anti-windup & reset : slpidlib/PID Controller  Controller=PI  Form=Parallel  TimeDomain=Discrete-time  UseExternalTs=off  SampleTime=-1  IntegratorMethod=Forward Euler  FilterMethod=Forward Euler  ControllerParametersSource=external  P=1  I=1  UseKiTs=on  D=0  UseExternalDerivativeSource=off  N=100  UseFilter=on  TunerSelectOption=Transfer Function Based (PID Tuner App)  InitialConditionSource=external  InitialConditionForIntegrator=0  InitialConditionForFilter=0  DifferentiatorICPrevScaledInput=0  ExternalReset=none  TrackingMode=off  Kt=1  LimitOutput=on  SatLimitsSource=internal  UpperSaturationLimit=0.8*inverter.V_dc*sqrt(3)/3  LowerSaturationLimit=-0.8*inverter.V_dc*sqrt(3)/3  LinearizeAsGain=on  AntiWindupMode=clamping  Kb=1  LimitIntegrator=off  UpperIntegratorSaturationLimit=inf  LowerIntegratorSaturationLimit=-inf  RndMeth=Simplest  POutMin=[]  POutMax=[]  IOutMin=[]  IOutMax=[]  DOutMin=[]  DOutMax=[]  NOutMin=[]  NOutMax=[]  SumOutMin=[]  SumOutMax=[]  SaturationOutDataTypeStr=Inherit: Inherit via back propagation  SaturationOutMin=[]  SaturationOutMax=[]  PParamMin=[]  PParamMax=[]  IParamMin=[]  IParamMax=[]  DParamMin=[]  DParamMax=[]  NParamMin=[]  NParamMax=[]  KbParamMin=[]  KbParamMax=[]  KtParamMin=[]  KtParamMax=[]  KbOutMin=[]  KbOutMax=[]  KtOutMin=[]  KtOutMax=[]  IntegratorOutMin=[]  IntegratorOutMax=[]  FilterOutMin=[]  FilterOutMax=[]  SumI1OutMin=[]  SumI1OutMax=[]  SumI2OutMin=[]  SumI2OutMax=[]  SumI3OutMin=[]  SumI3OutMax=[]  SumI4OutMin=[]  SumI4OutMax=[]  SumDOutMin=[]  SumDOutMax=[]  DifferentiatorOutMin=[]  DifferentiatorOutMax=[]  FilterDiffOutCoefMin=[]  FilterDiffOutCoefMax=[]  ReciprocalOutMin=[]  ReciprocalOutMax=[]  SumDenOutMin=[]  SumDenOutMax=[]  SumNumOutMin=[]  SumNumOutMax=[]  DivideOutMin=[]  DivideOutMax=[]  UdiffTsProdOutMin=[]  UdiffTsProdOutMax=[]  NTsProdOutMin=[]  NTsProdOutMax=[]  UintegralTsProdOutMin=[]  UintegralTsProdOutMax=[]  UngainTsProdOutMin=[]  UngainTsProdOutMax=[]  ClampingZeroOutDataTypeStr=Inherit: Inherit via back propagation  ClampingZeroOutMin=[]  ClampingZeroOutMax=[]  FilterDenConstantOutDataTypeStr=Inherit: Inherit via back propagation  FilterDenConstantOutMin=[]  FilterDenConstantOutMax=[]  PCopyOutDataTypeStr=Inherit: Inherit via back propagation  PCopyOutMin=[]  PCopyOutMax=[]  NCopyOutDataTypeStr=Inherit: Inherit via back propagation  NCopyOutMin=[]  NCopyOutMax=[]  IntegratorContinuousStateAttributes=''  IntegratorStateMustResolveToSignalObject=off  IntegratorRTWStateStorageClass=Auto  FilterContinuousStateAttributes=''  FilterStateMustResolveToSignalObject=off  FilterRTWStateStorageClass=Auto  ParallelPVariant=ExternalParameters  IdealPVariant=Disabled  IVariant=ExternalParameters  DVariant=Disabled  IntegratorVariant=Discrete  SatVariant=Enabled  AWVariant=DiscClampingParallel  PCopyVariant=Disabled  TRVariant=Disabled  FdbkBlocksVariant=Forward  IdealPFdbkVariant=Disabled  SatFdbkVariant=Disabled  DerivativeFilterVariant=Disabled  NVariant=Disabled  NCopyVariant=Disabled_SignalSpec  FilterICVariant=Disabled  IntegratorICVariant=ExternalICs  ExternalResetVariant=Disabled  TRSumVariant=Passthrough  SumFdbkVariant=Disabled  SumVariant=Sum_PI  TsampFilterVariant=InternalTs  TsampNgainVariant=Passthrough  TsampIntegralVariant=Disabled_SignalSpec  ExternalSaturationOutDataTypeStr=Inherit: Same as second input  DerivativeSourceVariant=Disabled  PreIntVariant=InternalPreInt
      settings: LibrarySourceBlock=mcbcontrolslib/PI Controller
  Sum : Sum  Inputs=|+-
  uQ_req : Outport
  wires:
  iQ_fdbk/1 -> Sum/2
  iQ_req/1 -> Sum/1
  Constant2/1 -> Discrete PI Controller with anti-windup & reset/2
  Constant1/1 -> Discrete PI Controller with anti-windup & reset/3
  Constant6/1 -> Discrete PI Controller with anti-windup & reset/4
  Discrete PI Controller with anti-windup & reset/1 -> uQ_req/1
  Sum/1 -> Discrete PI Controller with anti-windup & reset/1

== system FOCwithLOAD/Motor1 Speed control/Control_System/Closed Loop Control1/SVPWM/InvClark ==
  note: $i_a=i_\alpha\\ i_b=-\frac{1}{2}i_\alpha+\frac{\sqrt{3}}{2}i_\beta\\ i_c=-\frac{1}{2}i_\alpha-\frac{\sqrt{3}}{2}i_\beta$
  note: u_c_spwm
  note: u_b_spwm
  note: u_a_spwm
  u_alpha : Inport
  u_beta : Inport  Port=2
  Gain : Gain  Gain=-1/2
  Gain1 : Gain  Gain=sqrt(3)/2
  Mux : Mux  Inputs=3
  Sum : Sum  Inputs=|++
  Sum1 : Sum  Inputs=-+|
  u_abc_spwm : Outport
  wires:
  Mux/1 -> u_abc_spwm/1
  Sum1/1 -> Mux/3
  Sum/1 -> Mux/2
  u_alpha/1 -> Gain/1, Mux/1
  Gain1/1 -> Sum/2, Sum1/1
  u_beta/1 -> Gain1/1
  Gain/1 -> Sum/1, Sum1/2

== system FOCwithLOAD/Motor1 Speed control/Control_System/Closed Loop Control1/SVPWM/Sector Caculate ==
  Ualpha : Inport
  Ubeta : Inport  Port=2
  B0 : Fcn  Expr=u[2]
  B1 : Fcn  Expr=u[1]*sqrt(3/4)-0.5*u[2]
  B2 : Fcn  Expr=-u[1]*sqrt(3/4)-u[2]*0.5
  Constant : Constant
  Constant1 : Constant  Value=0
  Mux : Mux  Inputs=2
  Mux1 : Mux  Inputs=3
  N : Fcn  Expr=4*u[3]+2*u[2]+u[1]
  Switch : Switch  SaturateOnIntegerOverflow=off  InputSameDT=off
  Switch1 : Switch  SaturateOnIntegerOverflow=off  InputSameDT=off
  Switch2 : Switch  SaturateOnIntegerOverflow=off  InputSameDT=off
  "N " : Outport  VectorParamsAs1DForOutWhenUnconnected=off
  wires:
  Switch2/1 -> Mux1/3
  Switch/1 -> Mux1/1
  Ualpha/1 -> Mux/1
  Ubeta/1 -> Mux/2
  Mux/1 -> B2/1, B1/1, B0/1
  B0/1 -> Switch/2
  B1/1 -> Switch1/2
  B2/1 -> Switch2/2
  Constant/1 -> Switch/1, Switch2/1, Switch1/1
  Constant1/1 -> Switch/3, Switch1/3, Switch2/3
  Switch1/1 -> Mux1/2
  Mux1/1 -> N/1
  N/1 -> "N "/1

== system FOCwithLOAD/Motor1 Speed control/Control_System/Closed Loop Control1/SVPWM/T1T1 Caculate ==
  note: T1
  note: T2
  N : Inport
  XYZ : Inport  Port=2
  Tpwm : Inport  Port=3
  Demux : Demux  Outputs=3
  Fcn : Fcn  Expr=u(3)-u(2)-u(1)
  Fcn1 : Fcn  Expr=u(1)*u(3)/(u(1)+u(2))
  Fcn2 : Fcn  Expr=u(2)*u(3)/(u(1)+u(2))
  Gain : Gain  Gain=-1
  Gain1 : Gain  Gain=-1
  Gain2 : Gain  Gain=-1
  Multiport Switch : MultiPortSwitch  Inputs=6  SaturateOnIntegerOverflow=off  InputSameDT=off
  Multiport Switch1 : MultiPortSwitch  Inputs=6  SaturateOnIntegerOverflow=off  InputSameDT=off
  Mux : Mux  Inputs=3
  Switch : Switch  SaturateOnIntegerOverflow=off  InputSameDT=off
  Switch1 : Switch  Criteria=u2 > Threshold  SaturateOnIntegerOverflow=off  InputSameDT=off
  T1 : Outport  VectorParamsAs1DForOutWhenUnconnected=off
  T2 : Outport  Port=2  VectorParamsAs1DForOutWhenUnconnected=off
  wires:
  Tpwm/1 -> Mux/3
  XYZ/1 -> Demux/1
  Switch1/1 -> T2/1
  Switch/1 -> T1/1
  Fcn2/1 -> Switch1/3
  Fcn1/1 -> Switch/3
  Fcn/1 -> Switch/2, Switch1/2
  Mux/1 -> Fcn1/1, Fcn/1, Fcn2/1
  Multiport Switch/1 -> Switch/1, Mux/1
  Multiport Switch1/1 -> Switch1/1, Mux/2
  N/1 -> Multiport Switch/1, Multiport Switch1/1
  Demux/2 -> Multiport Switch/3, Multiport Switch1/2, Gain1/1
  Demux/3 -> Multiport Switch1/5, Multiport Switch/2, Gain2/1
  Demux/1 -> Multiport Switch/6, Multiport Switch1/4, Gain/1
  Gain/1 -> Multiport Switch1/3, Multiport Switch/5
  Gain2/1 -> Multiport Switch/4, Multiport Switch1/7
  Gain1/1 -> Multiport Switch1/6, Multiport Switch/7

== system FOCwithLOAD/Motor1 Speed control/Control_System/Closed Loop Control1/SVPWM/Tcm Caculate ==
  N : Inport
  T1 : Inport  Port=2
  T2 : Inport  Port=3
  Tpwm : Inport  Port=4
  Fcn : Fcn  Expr=(u[3]-u[1]-u[2])/4
  Fcn1 : Fcn  Expr=(u[3]+u[1]-u[2])/4
  Fcn2 : Fcn  Expr=(u[3]+u[2]+u[1])/4
  Multiport Switch : MultiPortSwitch  Inputs=6  SaturateOnIntegerOverflow=off  InputSameDT=off
  Multiport Switch1 : MultiPortSwitch  Inputs=6  SaturateOnIntegerOverflow=off  InputSameDT=off
  Multiport Switch2 : MultiPortSwitch  Inputs=6  SaturateOnIntegerOverflow=off  InputSameDT=off
  Mux : Mux  Inputs=3
  Mux1 : Mux  Inputs=3
  Tcm1 Tcm2 Tcm3 : Outport  VectorParamsAs1DForOutWhenUnconnected=off
  wires:
  Mux/1 -> Fcn2/1, Fcn/1, Fcn1/1
  Tpwm/1 -> Mux/3
  T2/1 -> Mux/2
  T1/1 -> Mux/1
  Multiport Switch2/1 -> Mux1/3
  Multiport Switch1/1 -> Mux1/2
  Multiport Switch/1 -> Mux1/1
  Mux1/1 -> Tcm1 Tcm2 Tcm3/1
  Fcn/1 -> Multiport Switch/3, Multiport Switch/4, Multiport Switch1/6, Multiport Switch2/5, Multiport Switch2/7, Multiport Switch1/2
  Fcn1/1 -> Multiport Switch1/5, Multiport Switch2/3, Multiport Switch2/6, Multiport Switch1/4, Multiport Switch/7, Multiport Switch/2
  Fcn2/1 -> Multiport Switch/5, Multiport Switch/6, Multiport Switch1/3, Multiport Switch1/7, Multiport Switch2/2, Multiport Switch2/4
  N/1 -> Multiport Switch2/1, Multiport Switch1/1, Multiport Switch/1

== system FOCwithLOAD/Motor1 Speed control/Control_System/Closed Loop Control1/SVPWM/XYZ Caculate ==
  Ualpha : Inport
  Ubeta : Inport  Port=2
  Ts : Inport  Port=3
  Udc : Inport  Port=4
  Add : Sum
  Add1 : Sum  Inputs=+-
  Gain : Gain  Gain=3/2
  Gain1 : Gain  Gain=sqrt(3)
  Gain2 : Gain  Gain=sqrt(3)/2
  Math Function : Math  Operator=reciprocal  SignedPower=on
  Mux : Mux  Inputs=3
  Product{,1..3} (4 alike) : Product  RndMeth=Zero
  XYZ : Outport  VectorParamsAs1DForOutWhenUnconnected=off
  wires:
  Mux/1 -> XYZ/1
  Product1/1 -> Mux/1
  Product3/1 -> Mux/2
  Product2/1 -> Mux/3
  Ualpha/1 -> Gain/1
  Ubeta/1 -> Gain2/1, Gain1/1
  Udc/1 -> Math Function/1
  Math Function/1 -> Product/2
  Ts/1 -> Product/1
  Gain1/1 -> Product1/1
  Product/1 -> Product2/2, Product1/2, Product3/2
  Gain/1 -> Add1/2, Add/2
  Gain2/1 -> Add/1, Add1/1
  Add1/1 -> Product2/1
  Add/1 -> Product3/1

== system FOCwithLOAD/Motor1 Speed control/Control_System/Closed Loop Control1/SVPWM/ei_t ==
  note: $e_i(t)=\frac{1}{2}(1-u^\ast_{max})+\frac{1}{2}(-1-u^\ast_{min})=-\frac{1}{2}(u^\ast_{max}+u^*_{min})$
  u_abc_spwm : Inport
  Demux : Demux  Outputs=3
  Gain : Gain  Gain=-1/2
  Max : MinMax  Function=max  Inputs=3
  Min : MinMax  Inputs=3
  Sum : Sum  Inputs=|++
  sit : Outport
  wires:
  Gain/1 -> sit/1
  Sum/1 -> Gain/1
  Max/1 -> Sum/2
  Min/1 -> Sum/1
  Demux/3 -> Min/3, Max/3
  Demux/2 -> Min/2, Max/2
  Demux/1 -> Min/1, Max/1
  u_abc_spwm/1 -> Demux/1

== system FOCwithLOAD/Motor1 Speed control/Control_System/Closed Loop Control1/Sample Choice/AB 采样计算2 ==
  Iabc : Inport
  AB : ActionPort  ActionPortLabel=else
  Demux : Demux  Outputs=3
  Mux : Mux  Inputs=3
  Sum : Sum  Inputs=--
  Terminator : Terminator
  IABC : Outport
  wires:
  Iabc/1 -> Demux/1
  Mux/1 -> IABC/1
  Demux/2 -> Sum/2, Mux/2
  Demux/1 -> Sum/1, Mux/1
  Sum/1 -> Mux/3
  Demux/3 -> Terminator/1

== system FOCwithLOAD/Motor1 Speed control/Control_System/Closed Loop Control1/Sample Choice/AC 采样计算1 ==
  Iabc : Inport
  AC : ActionPort  ActionPortLabel=elseif(u2 >= u1 & u2 >= u3)
  Demux : Demux  Outputs=3
  Mux : Mux  Inputs=3
  Sum : Sum  Inputs=|--
  Terminator : Terminator
  IABC : Outport
  wires:
  Demux/3 -> Mux/3, Sum/2
  Demux/1 -> Mux/1, Sum/1
  Iabc/1 -> Demux/1
  Mux/1 -> IABC/1
  Sum/1 -> Mux/2
  Demux/2 -> Terminator/1

== system FOCwithLOAD/Motor1 Speed control/Control_System/Closed Loop Control1/Sample Choice/BC 采样计算 ==
  Iabc : Inport
  选择BC : ActionPort  ActionPortLabel=if(u1 >= u2 & u1 >= u3)
  Demux : Demux  Outputs=3
  Mux : Mux  Inputs=3
  Sum : Sum  Inputs=|--
  Terminator : Terminator
  IABC : Outport
  wires:
  Iabc/1 -> Demux/1
  Demux/1 -> Terminator/1
  Mux/1 -> IABC/1
  Demux/2 -> Sum/1, Mux/2
  Demux/3 -> Mux/3, Sum/2
  Sum/1 -> Mux/1

== system FOCwithLOAD/Motor1 Speed control/Input Scaling/Calculate Phase Currents/Data_Type/Data_Type_Fixed_Point ==
  In1 : Inport
  Data Type Conversion : DataTypeConversion  OutDataTypeStr=fixdt(1,32,17)  ConvertRealWorld=Stored Integer (SI)  RndMeth=Simplest  SaturateOnIntegerOverflow=off
  Data Type Conversion1 : DataTypeConversion  OutDataTypeStr=dataType  RndMeth=Simplest  SaturateOnIntegerOverflow=off
  Q17 per unit conversion : ArithShift  BitShiftNumber=-6
  Iabc_meas_Real : Outport
  wires:
  In1/1 -> Q17 per unit conversion/1
  Data Type Conversion1/1 -> Iabc_meas_Real/1
  Data Type Conversion/1 -> Data Type Conversion1/1
  Q17 per unit conversion/1 -> Data Type Conversion/1

== system FOCwithLOAD/Motor1 Speed control/Input Scaling/Calculate Phase Currents/Data_Type/Data_Type_Float ==
  note: 电压值/（MOSFET导通值+采样电阻值）
  note: ADC值转电压值
  In1 : Inport
  Get ADC Voltage : Gain  Gain=target.ADC_Vref /target.ADC_MaxCount  OutDataTypeStr=dataType  RndMeth=Simplest
  Get Currents : Gain  Gain=1/inverter.ISenseVoltPerAmp  RndMeth=Simplest  OutDataTypeStr=Inherit: Same as input
  Iabc_meas_Real : Outport
  wires:
  Get ADC Voltage/1 -> Get Currents/1
  In1/1 -> Get ADC Voltage/1
  Get Currents/1 -> Iabc_meas_Real/1

== system FOCwithLOAD/Motor2 Torque control/Control_System/Closed Loop Control1/Controller/Filter ==
  R(n) : Inport
  Gain : Gain  Gain=1/(Tctr*innerPI.Filter.w0+1)
  Gain1 : Gain  Gain=(Tctr*innerPI.Filter.w0)/(Tctr*innerPI.Filter.w0+1)
  Sum : Sum  Inputs=|++
  Unit Delay : UnitDelay  SampleTime=-1  HasFrameUpgradeWarning=on
  Y(n) : Outport
  wires:
  Unit Delay/1 -> Gain/1  "Y(n-1)"
  Sum/1 -> Y(n)/1, Unit Delay/1  "Y(n)"
  Gain/1 -> Sum/2
  R(n)/1 -> Gain1/1
  Gain1/1 -> Sum/1
